simulink model "IMUsimulationsSimuLink"  (R2024b)
settings: Solver=VariableStepAuto  StartTime=0.0  StopTime=19000  RelTol=1e-3
settings Model: Creator=aramp  LastModifiedBy=aramp
settings SFSimCC: SimCustomHeaderCode="#include \"src/imu.hpp\""  SimUserIncludeDirs=src/  SimTargetLang=C++

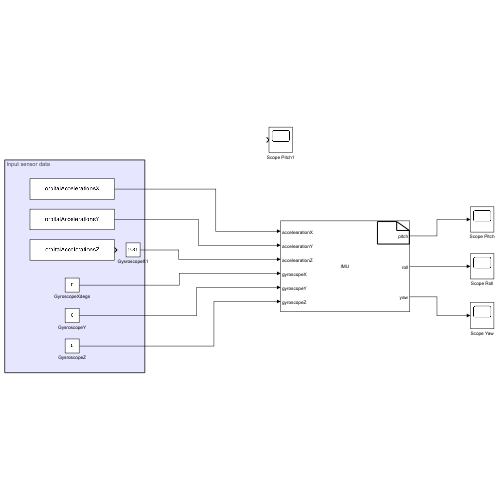
[thumbnail: Simulink's stored preview of the top-level diagram]
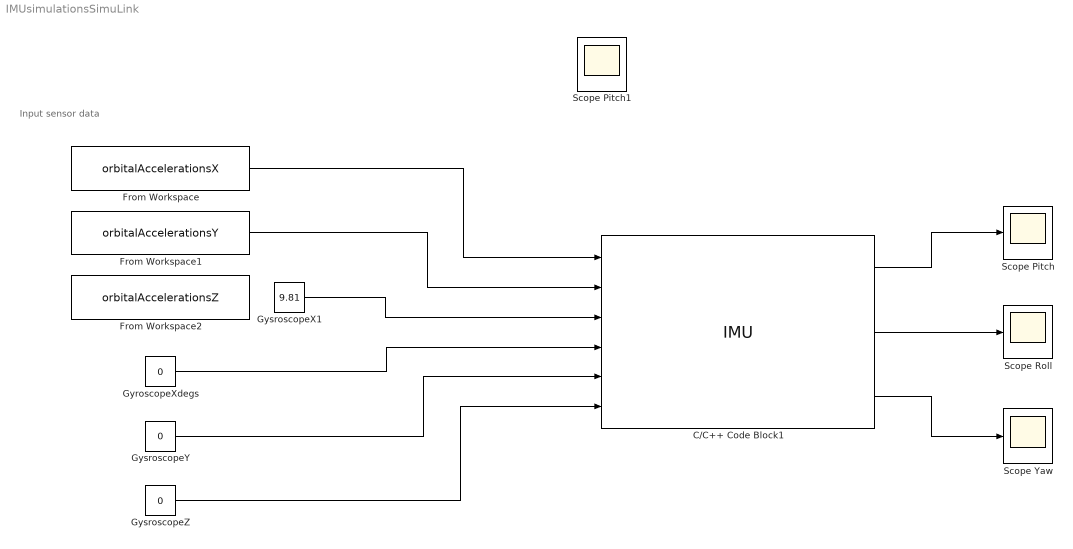
== system IMUsimulationsSimuLink ==
  note: Input sensor data
  C/C++ Code Block1 : S-Function  FunctionName=IMU  SFunctionModules=IMU_wrapper.cpp  SFunctionDeploymentMode=off  EnableBusSupport=off  mask(S-Function Builder){}
      mask help: Simulink:masks:SFunctionBuilder_MD
      mask init:
      | val = [[.9  0.75 0.75 1 1 .9 .9 1]',[1 1 0.75 0.75 .9 .9 1 .9]'];try , sys = get_param(gcb,'SfunBuilderFcnName');if isempty(sys), sys = get_param(gcb,'FunctionName'); end,catch, sys = get_param(gcb,'FunctionName'); end
      settings: CopyFcn=set_param(gcbh,'LinkStatus','none')  OpenFcn=sfunctionwizard(gcbh)
      mask Display:
      | plot(val(:,1),val(:,2))
      | disp(sys)
      | port_label('input',1,sprintf('%s', 'accelearationX'),'interpreter','tex')
      | port_label('input',2,sprintf('%s', 'accelearationY'),'interpreter','tex')
      | port_label('input',3,sprintf('%s', 'accelearationZ'),'interpreter','tex')
      | port_label('input',4,sprintf('%s', 'gyroscopeX'),'interpreter','tex')
      | port_label('input',5,sprintf('%s', 'gyroscopeY'),'interpreter','tex')
      | port_label('input',6,sprintf('%s', 'gyroscopeZ'),'interpreter','tex')
      | port_label('output',1,sprintf('%s', 'pitch'),'interpreter','tex')
      | port_label('output',2,sprintf('%s', 'roll'),'interpreter','tex')
      | port_label('output',3,sprintf('%s', 'yaw'),'interpreter','tex')
  From Workspace : FromWorkspace  VariableName=orbitalAccelerationsX  SampleTime=0.01
  From Workspace1 : FromWorkspace  VariableName=orbitalAccelerationsY  SampleTime=0.01
  From Workspace2 : FromWorkspace  VariableName=orbitalAccelerationsZ  SampleTime=0.01
  GyroscopeXdegs : Constant  Value=0
  GysroscopeX1 : Constant  Value=9.81
  GysroscopeY : Constant  Value=0
  GysroscopeZ : Constant  Value=0
  Scope Pitch : Scope
  Scope Pitch1 : Scope
  Scope Roll : Scope
  Scope Yaw : Scope
  wires:
  From Workspace1/1 -> C/C++ Code Block1/2
  C/C++ Code Block1/1 -> Scope Pitch/1
  C/C++ Code Block1/2 -> Scope Roll/1
  C/C++ Code Block1/3 -> Scope Yaw/1
  GyroscopeXdegs/1 -> C/C++ Code Block1/4
  GysroscopeY/1 -> C/C++ Code Block1/5
  GysroscopeZ/1 -> C/C++ Code Block1/6
  From Workspace/1 -> C/C++ Code Block1/1
  GysroscopeX1/1 -> C/C++ Code Block1/3
